simulink model "Full_Car_Model"  (R2023b)
settings: Solver=FixedStepAuto  StartTime=0.0  StopTime=t_end_sim  FixedStep=Ts_sim  RelTol=1e-3
values from neighbouring files (symbols this model uses):
  a_b_ref_sat = [ zeros(1,10) ... (first row only)    [A1_Init.m]    (also in C1_MonteCarloAnalysis.m)
  adaptive = 3    [A1_Init.m]    (also in C1_MonteCarloAnalysis.m = 1)
  data = A2_Full_car_model_parameters_4onBoard()    [A1_Init.m]    (also in C1_MonteCarloAnalysis.m)
  Ft_demand_F = [zeros(1,601) 200*ones(1,2400)]./data.R_F    [A1_Init.m]    (also in C1_MonteCarloAnalysis.m)
  Ft_demand_R = [zeros(1,(601-length(l_discr)))              200*ones(1,(2400+length(l_discr)))]./data.R_R    [A1_Init.m]    (also in C1_MonteCarloAnalysis.m)
  handmade_front = strcat(currentPath,'\Road_profiles\height_crg_files\','handmade_step_3cm_singlefunctions.crg')    [A1_Init.m]    (also in C1_MonteCarloAnalysis.m)
  handmade_mu_front = strcat(currentPath,'\Road_profiles\friction_crg_files\','handmade_fric_step_01_singlefunctions.crg')    [A1_Init.m]    (also in C1_MonteCarloAnalysis.m)
  handmade_mu_rear = handmade_mu_front    [A1_Init.m]    (also in C1_MonteCarloAnalysis.m)
  handmade_rear = handmade_front    [A1_Init.m]    (also in C1_MonteCarloAnalysis.m)
  LowLim_Q1 = -10    [A1_Init.m]    (also in C1_MonteCarloAnalysis.m)
  M = N    (= 10)    [A1_Init.m]    (also in C1_MonteCarloAnalysis.m)
  mu_distance = test_distance    [A1_Init.m]    (also in C1_MonteCarloAnalysis.m)
  mu_road = [ones(1,1001), 0.1*ones(1,2000)]    [A1_Init.m]    (also in C1_MonteCarloAnalysis.m)
  N = 10    [A1_Init.m]    (also in C1_MonteCarloAnalysis.m)
  N_iter = 3    [A1_Init.m]    (also in C1_MonteCarloAnalysis.m)
  omega_ini_F_L = x_u_dot_ini_F_L/data.R_F    [A1_Init.m]    (also in C1_MonteCarloAnalysis.m)
  omega_ini_F_R = x_u_dot_ini_R_R/data.R_F    [A1_Init.m]    (also in C1_MonteCarloAnalysis.m)
  omega_ini_R_L = x_u_dot_ini_R_L/data.R_R +2.483*1e-6    [A1_Init.m]    (also in C1_MonteCarloAnalysis.m)
  omega_ini_R_R = x_u_dot_ini_R_R/data.R_R+2.483*1e-6    [A1_Init.m]    (also in C1_MonteCarloAnalysis.m)
  passive = 2    [A1_Init.m]    (also in C1_MonteCarloAnalysis.m)
  Pitch = 0    [A1_Init.m]    (also in C1_MonteCarloAnalysis.m)
  Pitch_dot = 0    [A1_Init.m]    (also in C1_MonteCarloAnalysis.m)
  preview = 2    [A1_Init.m]    (also in C1_MonteCarloAnalysis.m)
  Q1 = 1e6    (= 1000000)    [A1_Init.m]    (also in C1_MonteCarloAnalysis.m)
  Q1_sat = 0    [A1_Init.m]    (also in C1_MonteCarloAnalysis.m)
  Q2 = 1e5    (= 100000)    [A1_Init.m]    (also in C1_MonteCarloAnalysis.m)
  QN1 = 0    [A1_Init.m]    (also in C1_MonteCarloAnalysis.m)
  QN2 = 0    [A1_Init.m]    (also in C1_MonteCarloAnalysis.m)
  R1 = 1e10    (= 10000000000)    [A1_Init.m]    (also in C1_MonteCarloAnalysis.m)
  r1_h0 = 0.99    [A1_Init.m]    (also in C1_MonteCarloAnalysis.m)
  r1_k = 1000    [A1_Init.m]    (also in C1_MonteCarloAnalysis.m)
  r1_max = 11    [A1_Init.m]    (also in C1_MonteCarloAnalysis.m)
  r1_min = -10    [A1_Init.m]    (also in C1_MonteCarloAnalysis.m)
  r2 = 2    [A1_Init.m]    (also in C1_MonteCarloAnalysis.m)
  R2 = 1e2    (= 100)    [A1_Init.m]    (also in C1_MonteCarloAnalysis.m)
  R2_rl = 2    [A1_Init.m]    (also in C1_MonteCarloAnalysis.m)
  road_profile = [zeros(1,801),ones(1,2200)*10*Step_selector]    [A1_Init.m]    (also in C1_MonteCarloAnalysis.m)
  T_distance = test_distance    [A1_Init.m]    (also in C1_MonteCarloAnalysis.m)
  T_hs_ini_F_L = 0    [A1_Init.m]    (also in C1_MonteCarloAnalysis.m)
  T_hs_ini_F_R = 0    [A1_Init.m]    (also in C1_MonteCarloAnalysis.m)
  T_hs_ini_R_L = 0    [A1_Init.m]    (also in C1_MonteCarloAnalysis.m)
  T_hs_ini_R_R = 0    [A1_Init.m]    (also in C1_MonteCarloAnalysis.m)
  test_distance = 0:0.01:30    [A1_Init.m]    (also in C1_MonteCarloAnalysis.m)
  theta_s_ini_F_L = 0    [A1_Init.m]    (also in C1_MonteCarloAnalysis.m)
  theta_s_ini_F_R = 0    [A1_Init.m]    (also in C1_MonteCarloAnalysis.m)
  theta_s_ini_R_L = 0    [A1_Init.m]    (also in C1_MonteCarloAnalysis.m)
  theta_s_ini_R_R = 0    [A1_Init.m]    (also in C1_MonteCarloAnalysis.m)
  theta_w_ini_F_L = -1.056*1e-2    (= -0.01056)    [A1_Init.m]    (also in C1_MonteCarloAnalysis.m)
  theta_w_ini_R_L = -1.056*1e-2    (= -0.01056)    [A1_Init.m]    (also in C1_MonteCarloAnalysis.m)
  Ts = 1e-3*[0 5 10 15 20 25 30 40 60 80 100]    [A1_Init.m]    (also in C1_MonteCarloAnalysis.m)
  w1_h0 = 0.0008    [A1_Init.m]    (also in C1_MonteCarloAnalysis.m)
  w1_k = 5000    [A1_Init.m]    (also in C1_MonteCarloAnalysis.m)
  w1_max = 9    [A1_Init.m]    (also in C1_MonteCarloAnalysis.m)
  w1_min = -10    [A1_Init.m]    (also in C1_MonteCarloAnalysis.m)
  w1_sat = 0.085    [A1_Init.m]    (also in C1_MonteCarloAnalysis.m)
  w2_h0 = 2    [A1_Init.m]    (also in C1_MonteCarloAnalysis.m)
  w2_inc = 0.05    [A1_Init.m]    (also in C1_MonteCarloAnalysis.m)
  w2_k = 10    [A1_Init.m]    (also in C1_MonteCarloAnalysis.m)
  w2_max = 5.3    [A1_Init.m]    (also in C1_MonteCarloAnalysis.m)
  w2_min = -10    [A1_Init.m]    (also in C1_MonteCarloAnalysis.m)
  Wmat_NMPC_init = [W(1,:) W(2,:) W(3,:) W(4,:)]    [A1_Init.m]    (also in C1_MonteCarloAnalysis.m)
  WNmat_NMPC_init = [WN(1,:) WN(2,:)]    [A1_Init.m]    (also in C1_MonteCarloAnalysis.m)
  X_0 = [z_b_dot_ini z_b_ini z_u_dot_ini_F_L z_u_ini_F_L x_b_dot_ini x_b_ini x_u_dot_ini_F_L x_u_ini_F_L          omega_ini_F_L theta_w_ini_F_L omega_ini_F_L theta_s_ini_F_L torque_ini_F_L]    [A1_Init.m]    (also in C1_MonteCarloAnalysis.m)
  x_b_dot_ini = speed_ini/3.6    (= 11.1111111111)    [A1_Init.m]    (also in C1_MonteCarloAnalysis.m)
  x_b_ini = data.b+pos_ini    [A1_Init.m]    (also in C1_MonteCarloAnalysis.m)
  x_u_dot_ini_F_L = speed_ini/3.6 - 1.125*1e-4    (= 11.1109986111)    [A1_Init.m]    (also in C1_MonteCarloAnalysis.m)
  x_u_dot_ini_F_R = speed_ini/3.6 - 1.125*1e-4    (= 11.1109986111)    [A1_Init.m]    (also in C1_MonteCarloAnalysis.m)
  x_u_dot_ini_R_L = speed_ini/3.6 - 1.125*1e-4    (= 11.1109986111)    [A1_Init.m]    (also in C1_MonteCarloAnalysis.m)
  x_u_dot_ini_R_R = speed_ini/3.6 - 1.125*1e-4    (= 11.1109986111)    [A1_Init.m]    (also in C1_MonteCarloAnalysis.m)
  x_u_ini_F_L = data.a+data.b+pos_ini    [A1_Init.m]    (also in C1_MonteCarloAnalysis.m)
  x_u_ini_F_R = data.a+data.b+pos_ini    [A1_Init.m]    (also in C1_MonteCarloAnalysis.m)
  x_u_ini_R_L = pos_ini    (= 0)    [A1_Init.m]    (also in C1_MonteCarloAnalysis.m)
  x_u_ini_R_R = pos_ini    (= 0)    [A1_Init.m]    (also in C1_MonteCarloAnalysis.m)
  z_b_dot_ini = 0    [A1_Init.m]    (also in C1_MonteCarloAnalysis.m)
  z_b_ini = 0    [A1_Init.m]    (also in C1_MonteCarloAnalysis.m)
  z_u_dot_ini_F_L = 0    [A1_Init.m]    (also in C1_MonteCarloAnalysis.m)
  z_u_dot_ini_F_R = 0    [A1_Init.m]    (also in C1_MonteCarloAnalysis.m)
  z_u_dot_ini_R_L = 0    [A1_Init.m]    (also in C1_MonteCarloAnalysis.m)
  z_u_dot_ini_R_R = 0    [A1_Init.m]    (also in C1_MonteCarloAnalysis.m)
  z_u_ini_F_L = 0    [A1_Init.m]    (also in C1_MonteCarloAnalysis.m)
  z_u_ini_F_R = 0    [A1_Init.m]    (also in C1_MonteCarloAnalysis.m)
  z_u_ini_R_L = 0    [A1_Init.m]    (also in C1_MonteCarloAnalysis.m)
  z_u_ini_R_R = 0    [A1_Init.m]    (also in C1_MonteCarloAnalysis.m)
undefined symbols (not defined in the file or in its folder): Delay_step, road_with_noise
libraries: mfswift_library x8, rllib x4, simulink x4
(part 4 of 7)

== system Full_Car_Model/PLANT MODEL WITH MF-SWIFT/REAR RIGHT WHEEL ==
  note: Rear rotational balance
  Tt_R_R : Inport
  BUS : Inport  Port=2
  Add1 : Sum
  Bus Creator : BusCreator  Inputs=3
  Bus Selector3 : BusSelector  OutputSignals=vertical_deflection,effective_rolling_radius,eff_plane_height,eff_plane_angle,longitudinal_slip,mu_x
  Clock1 : Clock
  Constant3 : Constant
  Demux1 : Demux  Outputs=2
  Gain3 : Gain  Gain=1/(data.I_y_R)
  Integrate velocity1 : Integrator  InitialCondition=theta_w_ini_R_L
  Integrate wheel acceleration : Integrator  InitialCondition=omega_ini_R_R
  MF-Swift : mfswift_library/MF-Swift  Tag=STI tyre  idtyre=2  tpfname=tir_name_R  rdfname=[handmade_rear,';',handmade_mu_rear];  road_mode=(2xxxx) opencrg  side_mode=(x3xxx) symmetric  cnt_mode=(xx5xx) enveloping  dyn_mode=(xxx3x) rigid-ring  mf_mode=(xxxx1) longitudinal  tv_model=Disabled  overwrite=off  use_mode=ISWITCH  internal_solver=off  enable_rr_init=on  optional_input=''  override_typarr=off  disp_debug=off
  "Select Fz, wheel" : Selector  InputPortWidth=3  IndexOptions=Index vector (dialog)  Indices=[1 3]  OutputSizes=[(-2)]
  Select My,wheel1 : Selector  InputPortWidth=3  IndexOptions=Index vector (dialog)  Indices=2  OutputSizes=[(-2)]
  Subsystem2 : Subsystem
  Subsystem5 : Subsystem
  Subsystem7 : Subsystem
  Terminator11 : Terminator
  Terminator13 : Terminator
  Terminator3 : Terminator
  To Workspace1 : ToWorkspace  VariableName=force_R_R  SampleTime=-1
  To Workspace4 : ToWorkspace  VariableName=torque_R_R  SampleTime=-1
  local2global : mfswift_library/local2global  Tag=local2global  init_pos=[0 0 (0.3833 - 0.5*data.m_total*9.81*data.a/data.L/data.k_t_R)]  init_angle=[0 0 0]
  Fx_R_R : Outport  VectorParamsAs1DForOutWhenUnconnected=off
  Fz_R_R_tot : Outport  Port=2  VectorParamsAs1DForOutWhenUnconnected=off
  Rotational_R_R : Outport  Port=3  VectorParamsAs1DForOutWhenUnconnected=off
  Slip_R_R : Outport  Port=4  VectorParamsAs1DForOutWhenUnconnected=off
  tag scope: mu_swift_R_R=global, w_swift_R_R=global
  wires:
  Demux1/1 -> Fx_R_R/1  "Fx_R_R"
  Bus Selector3/6 -> [mu_swift_R_R]  "<mu_x>"
  Bus Selector3/5 -> Slip_R_R/1  "<longitudinal_slip>"
  Gain3/1 -> Integrate wheel acceleration/1, Bus Creator/1  "omega_dot_R_R"
  Integrate wheel acceleration/1 -> Integrate velocity1/1, Bus Creator/2, MF-Swift/6  "omega_R_R"
  Bus Creator/1 -> Rotational_R_R/1
  Integrate velocity1/1 -> Bus Creator/3, MF-Swift/3  "theta_R_R"
  local2global/1 -> MF-Swift/1
  "Select Fz, wheel"/1 -> Demux1/1
  Tt_R_R/1 -> Add1/1
  Add1/1 -> Gain3/1
  Subsystem7/1(Road) -> MF-Swift/7  "With enveloping model i don't need this input"
  Bus Selector3/2 -> Terminator3/1  "<effective_rolling_radius>"
  MF-Swift/1 -> To Workspace1/1, "Select Fz, wheel"/1
  Constant3/1 -> Subsystem7/2(gain)
  Subsystem2/1(Velocity) -> local2global/1, MF-Swift/4
  MF-Swift/2 -> To Workspace4/1, Select My,wheel1/1
  MF-Swift/3 -> Bus Selector3/1
  Bus Selector3/1 -> Terminator13/1  "<vertical_deflection>"
  Demux1/2 -> Fz_R_R_tot/1
  Bus Selector3/4 -> Terminator11/1  "<eff_plane_angle>"
  Clock1/1 -> Subsystem7/1(time)
  local2global/2 -> MF-Swift/2
  Bus Selector3/3 -> [w_swift_R_R]  "<eff_plane_height>"
  Select My,wheel1/1 -> Add1/2
  Subsystem5/1(AngularVelocity) -> local2global/2, MF-Swift/5
  BUS/1 -> Subsystem2/1(speed), Subsystem5/1(Angular Speed)

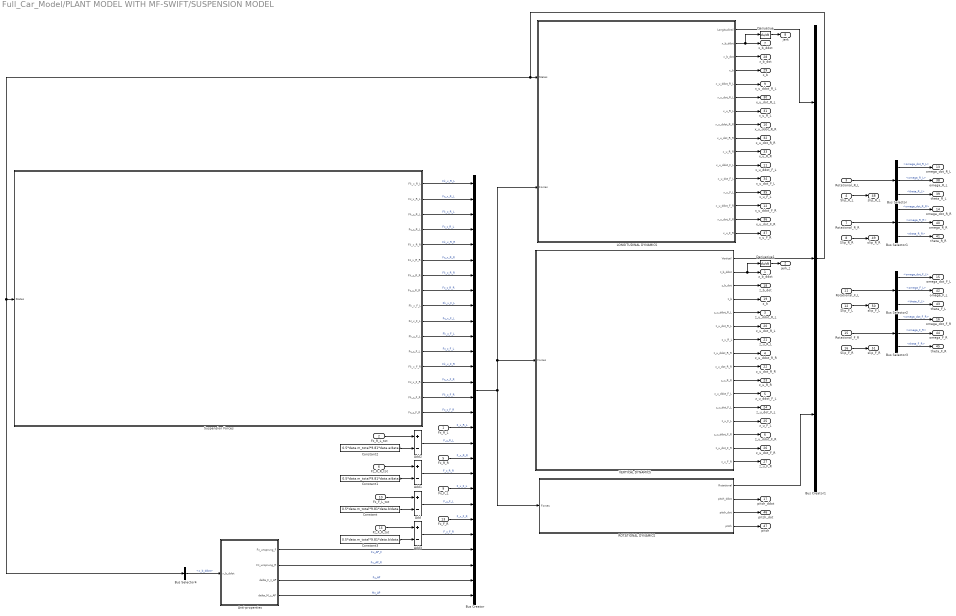
== system Full_Car_Model/PLANT MODEL WITH MF-SWIFT/SUSPENSION MODEL ==
  Fx_R_L : Inport
  Fz_R_L_tot : Inport  Port=2
  Rotational_R_L : Inport  Port=3
  Slip_R_L : Inport  Port=4
  Fx_R_R : Inport  Port=5
  Fz_R_R_tot : Inport  Port=6
  Rotational_R_R : Inport  Port=7
  Slip_R_R : Inport  Port=8
  Fx_F_L : Inport  Port=9
  Fz_F_L_tot : Inport  Port=10
  Rotational_F_L : Inport  Port=11
  Slip_F_L : Inport  Port=12
  Fx_F_R : Inport  Port=13
  Fz_F_R_tot : Inport  Port=14
  Rotational_F_R : Inport  Port=15
  Slip_F_R : Inport  Port=16
  Add{,1..3} (4 alike) : Sum  Inputs=+-
  Anti-properties : MATLAB Function  TreatAsAtomicUnit=on
  Bus Creator : BusCreator  Inputs=28
  Bus Creator1 : BusCreator  Inputs=3
  Bus Selector : BusSelector  OutputSignals=omega_dot_R_L,omega_R_L,theta_R_L
  Bus Selector1 : BusSelector  OutputSignals=omega_dot_R_R,omega_R_R,theta_R_R
  Bus Selector2 : BusSelector  OutputSignals=omega_dot_F_L,omega_F_L,theta_F_L
  Bus Selector3 : BusSelector  OutputSignals=omega_dot_F_R,omega_F_R,theta_F_R
  Bus Selector4 : BusSelector  OutputSignals=Longitudinal.x_b_ddot
  Constant : Constant  Value=0.5*data.m_total*9.81*data.b/data.L
  Constant1 : Constant  Value=0.5*data.m_total*9.81*data.a/data.L
  Constant2 : Constant  Value=0.5*data.m_total*9.81*data.a/data.L
  Constant3 : Constant  Value=0.5*data.m_total*9.81*data.b/data.L
  Derivative : Derivative
  Derivative1 : Derivative
  LONGITUDINAL DYNAMICS : Subsystem
  ROTATIONAL DYNAMICS : Subsystem
  Suspension Forces : Subsystem
  VERTICAL DYNAMICS : Subsystem
  z_b_ddot : Outport
  jerk_z : Outport  Port=2
  z_u_ddot_R_L : Outport  Port=3
  z_u_ddot_R_R : Outport  Port=4
  z_u_ddot_F_L : Outport  Port=5
  z_u_ddot_F_R : Outport  Port=6
  x_b_ddot : Outport  Port=7
  jerk : Outport  Port=8
  x_u_ddot_R_L : Outport  Port=9
  x_u_ddot_R_R : Outport  Port=10
  x_u_ddot_F_L : Outport  Port=11
  x_u_ddot_F_R : Outport  Port=12
  omega_dot_R_L : Outport  Port=13
  omega_dot_R_R : Outport  Port=14
  omega_dot_F_L : Outport  Port=15
  omega_dot_F_R : Outport  Port=16
  pitch_ddot : Outport  Port=17
  z_b_dot : Outport  Port=18
  z_b : Outport  Port=19
  z_u_dot_R_L : Outport  Port=20
  z_u_R_L : Outport  Port=21
  z_u_dot_R_R : Outport  Port=22
  z_u_R_R : Outport  Port=23
  z_u_dot_F_L : Outport  Port=24
  z_u_F_L : Outport  Port=25
  z_u_dot_F_R : Outport  Port=26
  z_u_F_R : Outport  Port=27
  x_b_dot : Outport  Port=28
  x_b : Outport  Port=29
  x_u_dot_R_L : Outport  Port=30
  x_u_R_L : Outport  Port=31
  x_u_dot_R_R : Outport  Port=32
  x_u_R_R : Outport  Port=33
  x_u_dot_F_L : Outport  Port=34
  x_u_F_L : Outport  Port=35
  x_u_dot_F_R : Outport  Port=36
  x_u_F_R : Outport  Port=37
  omega_R_L : Outport  Port=38
  theta_R_L : Outport  Port=39
  omega_R_R : Outport  Port=40
  theta_R_R : Outport  Port=41
  omega_F_L : Outport  Port=42
  theta_F_L : Outport  Port=43
  omega_F_R : Outport  Port=44
  theta_F_R : Outport  Port=45
  pitch_dot : Outport  Port=46
  pitch : Outport  Port=47
  slip_R_L : Outport  Port=48
  slip_R_R : Outport  Port=49
  slip_F_L : Outport  Port=50
  slip_F_R : Outport  Port=51
  wires:
  Anti-properties/2(Fz_unsprung_R) -> Bus Creator/26  "Fu_AP_R"
  Bus Selector4/1 -> Anti-properties/1(x_b_ddot)  "<x_b_ddot>"
  Anti-properties/4(delta_M_z_AP) -> Bus Creator/28  "Mz_AP"
  Anti-properties/3(delta_F_z_AP) -> Bus Creator/27  "Fz_AP"
  Anti-properties/1(Fz_unsprung_F) -> Bus Creator/25  "Fu_AP_F"
  Bus Creator1/1 -> LONGITUDINAL DYNAMICS/1(States), Suspension Forces/1(States), Bus Selector4/1
  Derivative1/1 -> jerk_z/1
  Derivative/1 -> jerk/1
  Slip_F_R/1 -> slip_F_R/1
  Bus Selector3/1 -> omega_dot_F_R/1  "<omega_dot_F_R>"
  Bus Selector3/2 -> omega_F_R/1  "<omega_F_R>"
  Bus Selector3/3 -> theta_F_R/1  "<theta_F_R>"
  Slip_F_L/1 -> slip_F_L/1
  Bus Selector2/3 -> theta_F_L/1  "<theta_F_L>"
  Bus Selector2/2 -> omega_F_L/1  "<omega_F_L>"
  Bus Selector2/1 -> omega_dot_F_L/1  "<omega_dot_F_L>"
  Slip_R_R/1 -> slip_R_R/1
  Bus Selector1/1 -> omega_dot_R_R/1  "<omega_dot_R_R>"
  Bus Selector1/2 -> omega_R_R/1  "<omega_R_R>"
  Bus Selector1/3 -> theta_R_R/1  "<theta_R_R>"
  Slip_R_L/1 -> slip_R_L/1
  Bus Selector/3 -> theta_R_L/1  "<theta_R_L>"
  Bus Selector/2 -> omega_R_L/1  "<omega_R_L>"
  Bus Selector/1 -> omega_dot_R_L/1  "<omega_dot_R_L>"
  Rotational_F_R/1 -> Bus Selector3/1
  Rotational_F_L/1 -> Bus Selector2/1
  Rotational_R_R/1 -> Bus Selector1/1
  Rotational_R_L/1 -> Bus Selector/1
  VERTICAL DYNAMICS/2(z_b_ddot) -> z_b_ddot/1, Derivative1/1
  VERTICAL DYNAMICS/3(z_b_dot) -> z_b_dot/1
  VERTICAL DYNAMICS/7(z_u_R_L) -> z_u_R_L/1
  VERTICAL DYNAMICS/6(z_u_dot_R_L) -> z_u_dot_R_L/1
  VERTICAL DYNAMICS/5(z_u_ddot_R_L) -> z_u_ddot_R_L/1
  VERTICAL DYNAMICS/4(z_b) -> z_b/1
  VERTICAL DYNAMICS/10(z_u_R_R) -> z_u_R_R/1
  VERTICAL DYNAMICS/11(z_u_ddot_F_L) -> z_u_ddot_F_L/1
  VERTICAL DYNAMICS/12(z_u_dot_F_L) -> z_u_dot_F_L/1
  VERTICAL DYNAMICS/13(z_u_F_L) -> z_u_F_L/1
  VERTICAL DYNAMICS/9(z_u_dot_R_R) -> z_u_dot_R_R/1
  VERTICAL DYNAMICS/8(z_u_ddot_R_R) -> z_u_ddot_R_R/1
  VERTICAL DYNAMICS/16(z_u_F_R) -> z_u_F_R/1
  VERTICAL DYNAMICS/15(z_u_dot_F_R) -> z_u_dot_F_R/1
  VERTICAL DYNAMICS/14(z_u_ddot_F_R) -> z_u_ddot_F_R/1
  ROTATIONAL DYNAMICS/2(pitch_ddot) -> pitch_ddot/1
  ROTATIONAL DYNAMICS/4(pitch) -> pitch/1
  ROTATIONAL DYNAMICS/3(pitch_dot) -> pitch_dot/1
  LONGITUDINAL DYNAMICS/14(x_u_ddot_F_R) -> x_u_ddot_F_R/1
  LONGITUDINAL DYNAMICS/15(x_u_dot_F_R) -> x_u_dot_F_R/1
  LONGITUDINAL DYNAMICS/16(x_u_F_R) -> x_u_F_R/1
  LONGITUDINAL DYNAMICS/8(x_u_ddot_R_R) -> x_u_ddot_R_R/1
  LONGITUDINAL DYNAMICS/9(x_u_dot_R_R) -> x_u_dot_R_R/1
  LONGITUDINAL DYNAMICS/13(x_u_F_L) -> x_u_F_L/1
  LONGITUDINAL DYNAMICS/12(x_u_dot_F_L) -> x_u_dot_F_L/1
  LONGITUDINAL DYNAMICS/11(x_u_ddot_F_L) -> x_u_ddot_F_L/1
  LONGITUDINAL DYNAMICS/10(x_u_R_R) -> x_u_R_R/1
  LONGITUDINAL DYNAMICS/4(x_b) -> x_b/1
  LONGITUDINAL DYNAMICS/5(x_u_ddot_R_L) -> x_u_ddot_R_L/1
  LONGITUDINAL DYNAMICS/6(x_u_dot_R_L) -> x_u_dot_R_L/1
  LONGITUDINAL DYNAMICS/7(x_u_R_L) -> x_u_R_L/1
  LONGITUDINAL DYNAMICS/3(x_b_dot) -> x_b_dot/1
  LONGITUDINAL DYNAMICS/2(x_b_ddot) -> x_b_ddot/1, Derivative/1
  ROTATIONAL DYNAMICS/1(Rotational) -> Bus Creator1/3
  VERTICAL DYNAMICS/1(Vertical) -> Bus Creator1/2
  LONGITUDINAL DYNAMICS/1(Longitudinal) -> Bus Creator1/1
  Bus Creator/1 -> ROTATIONAL DYNAMICS/1(Forces), LONGITUDINAL DYNAMICS/2(Forces), VERTICAL DYNAMICS/1(Forces)
  Suspension Forces/2(Fc_x_R_L) -> Bus Creator/2  "Fc_x_R_L"
  Suspension Forces/3(Fk_z_R_L) -> Bus Creator/3  "Fk_z_R_L"
  Suspension Forces/4(Fc_z_R_L) -> Bus Creator/4  "Fc_z_R_L"
  Suspension Forces/5(Fk_x_R_R) -> Bus Creator/5  "Fk_x_R_R"
  Suspension Forces/6(Fc_x_R_R) -> Bus Creator/6  "Fc_x_R_R"
  Suspension Forces/7(Fk_z_R_R) -> Bus Creator/7  "Fk_z_R_R"
  Suspension Forces/8(Fc_z_R_R) -> Bus Creator/8  "Fc_z_R_R"
  Suspension Forces/9(Fk_x_F_L) -> Bus Creator/9  "Fk_x_F_L"
  Suspension Forces/10(Fc_x_F_L) -> Bus Creator/10  "Fc_x_F_L"
  Suspension Forces/11(Fk_z_F_L) -> Bus Creator/11  "Fk_z_F_L"
  Suspension Forces/12(Fc_z_F_L) -> Bus Creator/12  "Fc_z_F_L"
  Suspension Forces/13(Fk_x_F_R) -> Bus Creator/13  "Fk_x_F_R"
  Suspension Forces/14(Fc_x_F_R) -> Bus Creator/14  "Fc_x_F_R"
  Suspension Forces/15(Fk_z_F_R) -> Bus Creator/15  "Fk_z_F_R"
  Suspension Forces/16(Fc_z_F_R) -> Bus Creator/16  "Fc_z_F_R"
  Suspension Forces/1(Fk_x_R_L) -> Bus Creator/1  "Fk_x_R_L"
  Constant3/1 -> Add3/2
  Fz_F_R_tot/1 -> Add3/1
  Add3/1 -> Bus Creator/24  "F_z_F_R"
  Add1/1 -> Bus Creator/20  "F_z_R_R"
  Constant1/1 -> Add1/2
  Fz_R_R_tot/1 -> Add1/1
  Add2/1 -> Bus Creator/18  "F_z_R_L"
  Constant2/1 -> Add2/2
  Fz_R_L_tot/1 -> Add2/1
  Add/1 -> Bus Creator/22  "F_z_F_L"
  Constant/1 -> Add/2
  Fz_F_L_tot/1 -> Add/1
  Fx_R_L/1 -> Bus Creator/17  "F_x_R_L"
  Fx_R_R/1 -> Bus Creator/19  "F_x_R_R"
  Fx_F_L/1 -> Bus Creator/21  "F_x_F_L"
  Fx_F_R/1 -> Bus Creator/23  "F_x_F_R"

== system Full_Car_Model/CONTROLLER FRONT LEFT/RL_weights/Subsystem2 ==
  Online Data : Inport
  Delay : Delay  Commented=on  DelayLength=1  SampleTime=Ts(2)
  MATLAB Function : MATLAB Function  TreatAsAtomicUnit=on
  Memory{,1..4} (5 alike) : Memory  InheritSampleTime=on
  Mux : Mux  Inputs=5
  Mux2 : Mux  Inputs=2
  Selector : Selector  NumberOfDimensions=2  InputPortWidth=1  IndexOptions=Index vector (dialog),Select all  Indices=1,1  OutputSizes=1,1
  Selector1 : Selector  NumberOfDimensions=2  InputPortWidth=1  IndexOptions=Index vector (dialog),Select all  Indices=1,1  OutputSizes=1,1
  w_prev : Outport
  mu_act_prev : Outport  Port=2
  sigma_ref_act : Outport  Port=3
  wires:
  Online Data/1 -> MATLAB Function/1(OnlineData)
  MATLAB Function/1(w) -> Mux2/2, Selector/1
  Selector/1 -> Memory/1  "w1"
  Memory/1 -> Memory1/1, Mux/5
  Memory1/1 -> Memory2/1, Mux/4
  Memory2/1 -> Memory3/1, Mux/3
  Memory3/1 -> Memory4/1, Mux/2
  Memory4/1 -> Mux/1
  Mux/1 -> Mux2/1
  Mux2/1 -> w_prev/1
  MATLAB Function/2(mu_act) -> mu_act_prev/1
  MATLAB Function/3(sigma_ref) -> Selector1/1
  Selector1/1 -> sigma_ref_act/1

== system Full_Car_Model/CONTROLLER FRONT LEFT/ROAD PREVIEW/Time-based Road Preview ==
  note: Absolute longitudinal wheel position along t_h
      | (assuming contant speed along t_h)
  x_u : Inport
  x_u_dot : Inport  Port=2
  1-D Lookup Table : Lookup_n-D  NumberOfTableDimensions=1  BreakpointsForDimension1=mu_distance  Table=mu_road  InternalRulePriority=Speed  RndMeth=Simplest
  Delay1 : Delay  Commented=on  DelayLength=Delay_step
  Gain1 : Gain  Gain=1e-3
  MATLAB Function1 : MATLAB Function  TreatAsAtomicUnit=on
  MATLAB Function4 : MATLAB Function  TreatAsAtomicUnit=on
  MATLAB Function5 : MATLAB Function  TreatAsAtomicUnit=on
  To Workspace : ToWorkspace  VariableName=roadprofile_front_plot  SaveFormat=Timeseries  SampleTime=-1
  X(i)1 : MATLAB Function  TreatAsAtomicUnit=on
  Z_road with noise2 : Lookup_n-D  Commented=on  NumberOfTableDimensions=1  BreakpointsForDimension1=test_distance  Table=road_with_noise  InterpMethod=Flat  InternalRulePriority=Speed  RndMeth=Simplest
  Z_road1 : Lookup_n-D  NumberOfTableDimensions=1  BreakpointsForDimension1=test_distance  Table=road_profile  InterpMethod=Flat  InternalRulePriority=Speed  RndMeth=Simplest
  Z_road2 : Lookup_n-D  NumberOfTableDimensions=1  BreakpointsForDimension1=test_distance  Table=road_profile  InterpMethod=Flat  InternalRulePriority=Speed  RndMeth=Simplest
  w : Outport
  beta_y : Outport  Port=2
  mu_prev : Outport  Port=3
  wires:
  Z_road2/1 -> To Workspace/1
  MATLAB Function1/1(Z_ef) -> MATLAB Function4/1(Z_ef)
  MATLAB Function1/2(Z_er) -> MATLAB Function4/2(Z_er)
  1-D Lookup Table/1 -> mu_prev/1
  X(i)1/1(X_i) -> 1-D Lookup Table/1, MATLAB Function5/1(X_i)  "X(i)"
  Gain1/1 -> MATLAB Function1/1(z_road)
  MATLAB Function4/1(w) -> w/1
  Z_road1/1 -> Gain1/1
  MATLAB Function5/1(X_road) -> Z_road1/1
  x_u/1 -> X(i)1/1(X_u_current), Z_road2/1
  x_u_dot/1 -> X(i)1/2(x_u_dot_current)
  MATLAB Function4/2(beta_y) -> beta_y/1

== system Full_Car_Model/CONTROLLER FRONT LEFT/Rule based/Flag ==
  Measurement data : Inport
  mu_prev : Inport  Port=2
  Add : Sum  Inputs=+-
  Bus Selector : BusSelector  OutputSignals=Accelerations.x_b_ddot
  Constant : Constant  Value=0.5*data.m_total*data.g*data.b/data.L
  Gain : Gain  Gain=0.5*data.m_total*data.hg/data.L
  Gain1 : Gain  Gain=0.6
  GreaterThan : RelationalOperator  Operator=>  OutDataTypeStr=boolean  RndMeth=Simplest  InputSameDT=off
  Memory : Memory
  OR : Logic  Operator=OR  Inputs=1  IconShape=distinctive  AllPortsSameDT=off  OutDataTypeStr=boolean
  Product : Product
  Flag : Outport
  wires:
  Constant/1 -> Add/1
  Bus Selector/1 -> Memory/1  "<x_b_ddot>"
  [Ft_req_F] -> GreaterThan/1
  Gain/1 -> Add/2
  Add/1 -> Product/1
  Measurement data/1 -> Bus Selector/1
  GreaterThan/1 -> OR/1
  Product/1 -> Gain1/1
  Memory/1 -> Gain/1
  mu_prev/1 -> Product/2
  Gain1/1 -> GreaterThan/2
  OR/1 -> Flag/1

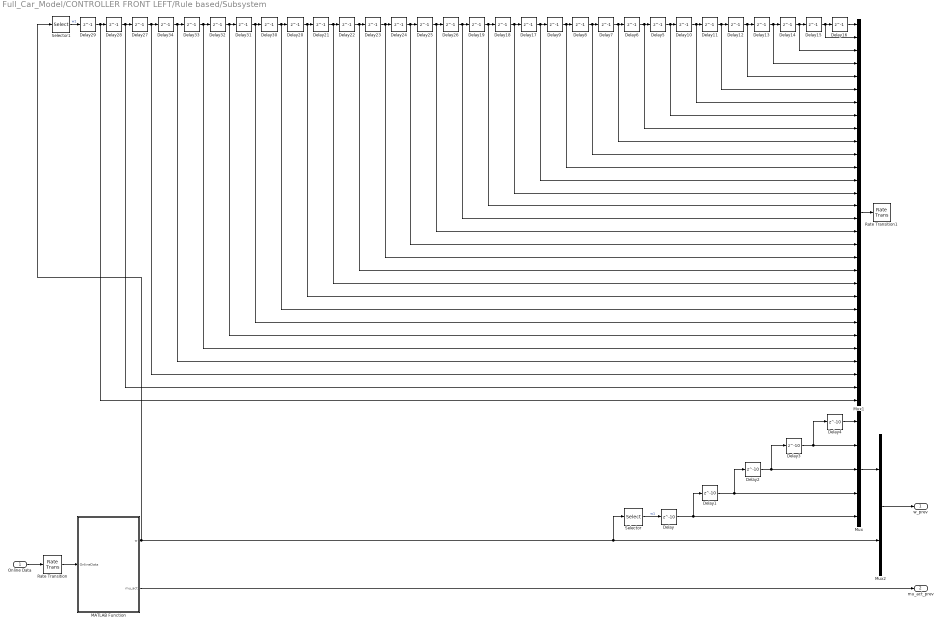
== system Full_Car_Model/CONTROLLER FRONT LEFT/Rule based/Subsystem ==
  Online Data : Inport
  Delay{,1..4} (5 alike) : Delay  DelayLength=10
  Delay{5..34} (30 alike) : Delay  DelayLength=1
  MATLAB Function : MATLAB Function  TreatAsAtomicUnit=on
  Mux : Mux  Inputs=5
  Mux1 : Mux  Inputs=30
  Mux2 : Mux  Inputs=2
  Rate Transition : RateTransition  OutPortSampleTime=Ts(2)
  Rate Transition1 : RateTransition  OutPortSampleTime=Ts(2)
  Selector : Selector  NumberOfDimensions=2  InputPortWidth=1  IndexOptions=Index vector (dialog),Select all  Indices=1,1  OutputSizes=1,1
  Selector1 : Selector  NumberOfDimensions=2  InputPortWidth=1  IndexOptions=Index vector (dialog),Select all  Indices=1,1  OutputSizes=1,1
  w_prev : Outport
  mu_act_prev : Outport  Port=2
  wires:
  MATLAB Function/1(w) -> Mux2/2, Selector/1, Selector1/1
  MATLAB Function/2(mu_act) -> mu_act_prev/1
  Mux1/1 -> Rate Transition1/1
  Rate Transition/1 -> MATLAB Function/1(OnlineData)
  Mux2/1 -> w_prev/1
  Delay4/1 -> Mux/1
  Delay3/1 -> Delay4/1, Mux/2
  Delay2/1 -> Delay3/1, Mux/3
  Delay1/1 -> Mux/4, Delay2/1
  Delay/1 -> Mux/5, Delay1/1
  Selector/1 -> Delay/1  "w1"
  Online Data/1 -> Rate Transition/1
  Delay5/1 -> Mux1/8, Delay10/1
  Selector1/1 -> Delay29/1  "w1"
  Delay10/1 -> Mux1/7, Delay11/1
  Delay11/1 -> Mux1/6, Delay12/1
  Delay12/1 -> Mux1/5, Delay13/1
  Delay13/1 -> Mux1/4, Delay14/1
  Delay14/1 -> Mux1/3, Delay15/1
  Delay15/1 -> Mux1/2, Delay16/1
  Delay16/1 -> Mux1/1
  Delay6/1 -> Mux1/9, Delay5/1
  Delay7/1 -> Mux1/10, Delay6/1
  Delay8/1 -> Delay7/1, Mux1/11
  Delay9/1 -> Mux1/12, Delay8/1
  Delay17/1 -> Mux1/13, Delay9/1
  Delay18/1 -> Mux1/14, Delay17/1
  Delay19/1 -> Delay18/1, Mux1/15
  Delay26/1 -> Mux1/16, Delay19/1
  Delay25/1 -> Mux1/17, Delay26/1
  Delay24/1 -> Mux1/18, Delay25/1
  Delay22/1 -> Mux1/20, Delay23/1
  Delay34/1 -> Mux1/27, Delay33/1
  Delay33/1 -> Mux1/26, Delay32/1
  Delay31/1 -> Mux1/24, Delay30/1
  Delay32/1 -> Mux1/25, Delay31/1
  Delay30/1 -> Mux1/23, Delay20/1
  Delay28/1 -> Mux1/29, Delay27/1
  Delay27/1 -> Mux1/28, Delay34/1
  Delay23/1 -> Mux1/19, Delay24/1
  Delay21/1 -> Mux1/21, Delay22/1
  Delay29/1 -> Mux1/30, Delay28/1
  Delay20/1 -> Mux1/22, Delay21/1
  Mux/1 -> Mux2/1

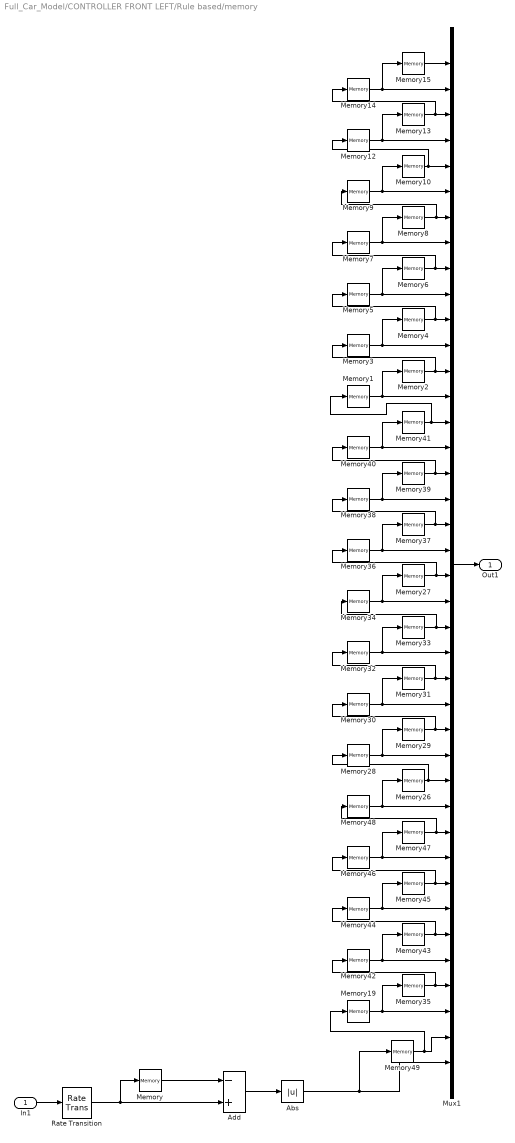
== system Full_Car_Model/CONTROLLER FRONT LEFT/Rule based/memory ==
  In1 : Inport
  Abs : Abs  SaturateOnIntegerOverflow=off
  Add : Sum  Inputs=-+
  Memory{,1..10,12..15,19,26..49} (40 alike) : Memory  InheritSampleTime=on
  Mux1 : Mux  Inputs=40
  Rate Transition : RateTransition  OutPortSampleTime=Ts(2)
  Out1 : Outport
  wires:
  Abs/1 -> Mux1/40, Memory49/1
  Memory49/1 -> Mux1/39, Memory19/1
  Memory19/1 -> Memory35/1, Mux1/38
  Memory47/1 -> Memory48/1, Mux1/31
  Memory42/1 -> Memory43/1, Mux1/36
  Memory44/1 -> Memory45/1, Mux1/34
  Memory43/1 -> Memory44/1, Mux1/35
  Memory33/1 -> Memory34/1, Mux1/23
  Memory46/1 -> Memory47/1, Mux1/32
  Memory32/1 -> Memory33/1, Mux1/24
  Memory38/1 -> Memory39/1, Mux1/18
  Memory48/1 -> Memory26/1, Mux1/30
  Memory45/1 -> Memory46/1, Mux1/33
  Memory30/1 -> Memory31/1, Mux1/26
  Memory26/1 -> Memory28/1, Mux1/29
  Memory37/1 -> Memory38/1, Mux1/19
  Memory29/1 -> Memory30/1, Mux1/27
  Memory31/1 -> Memory32/1, Mux1/25
  Memory27/1 -> Memory36/1, Mux1/21
  Memory28/1 -> Memory29/1, Mux1/28
  Memory34/1 -> Memory27/1, Mux1/22
  Memory40/1 -> Memory41/1, Mux1/16
  Memory41/1 -> Mux1/15, Memory1/1
  Memory39/1 -> Memory40/1, Mux1/17
  Memory35/1 -> Memory42/1, Mux1/37
  Memory36/1 -> Memory37/1, Mux1/20
  Add/1 -> Abs/1
  In1/1 -> Rate Transition/1
  Memory/1 -> Add/1
  Rate Transition/1 -> Add/2, Memory/1
  Memory14/1 -> Memory15/1, Mux1/2
  Memory12/1 -> Memory13/1, Mux1/4
  Memory15/1 -> Mux1/1
  Memory13/1 -> Memory14/1, Mux1/3
  Memory10/1 -> Mux1/5, Memory12/1
  Memory9/1 -> Memory10/1, Mux1/6
  Memory8/1 -> Memory9/1, Mux1/7
  Memory7/1 -> Memory8/1, Mux1/8
  Memory6/1 -> Memory7/1, Mux1/9
  Memory5/1 -> Memory6/1, Mux1/10
  Memory4/1 -> Mux1/11, Memory5/1
  Memory3/1 -> Memory4/1, Mux1/12
  Memory2/1 -> Mux1/13, Memory3/1
  Memory1/1 -> Memory2/1, Mux1/14
  Mux1/1 -> Out1/1

== system Full_Car_Model/CONTROLLER FRONT RIGHT/RL_weights/Subsystem2 ==
  Online Data : Inport
  Delay : Delay  Commented=on  DelayLength=1  SampleTime=Ts(2)
  MATLAB Function : MATLAB Function  TreatAsAtomicUnit=on
  Memory{,1..4} (5 alike) : Memory  InheritSampleTime=on
  Mux : Mux  Inputs=5
  Mux2 : Mux  Inputs=2
  Selector : Selector  NumberOfDimensions=2  InputPortWidth=1  IndexOptions=Index vector (dialog),Select all  Indices=1,1  OutputSizes=1,1
  Selector1 : Selector  NumberOfDimensions=2  InputPortWidth=1  IndexOptions=Index vector (dialog),Select all  Indices=1,1  OutputSizes=1,1
  w_prev : Outport
  mu_act_prev : Outport  Port=2
  sigma_ref_act : Outport  Port=3
  wires:
  Online Data/1 -> MATLAB Function/1(OnlineData)
  MATLAB Function/1(w) -> Mux2/2, Selector/1
  Selector/1 -> Memory/1  "w1"
  Memory/1 -> Memory1/1, Mux/5
  Memory1/1 -> Memory2/1, Mux/4
  Memory2/1 -> Memory3/1, Mux/3
  Memory3/1 -> Memory4/1, Mux/2
  Memory4/1 -> Mux/1
  Mux/1 -> Mux2/1
  Mux2/1 -> w_prev/1
  MATLAB Function/2(mu_act) -> mu_act_prev/1
  MATLAB Function/3(sigma_ref) -> Selector1/1
  Selector1/1 -> sigma_ref_act/1

== system Full_Car_Model/CONTROLLER FRONT RIGHT/ROAD PREVIEW/Time-based Road Preview ==
  note: Absolute longitudinal wheel position along t_h
      | (assuming contant speed along t_h)
  x_u : Inport
  x_u_dot : Inport  Port=2
  1-D Lookup Table : Lookup_n-D  NumberOfTableDimensions=1  BreakpointsForDimension1=mu_distance  Table=mu_road  InternalRulePriority=Speed  RndMeth=Simplest
  Delay1 : Delay  Commented=on  DelayLength=Delay_step
  Demux5 : Demux  Commented=on  Outputs=6
  Demux6 : Demux  Commented=on  Outputs=6
  Gain1 : Gain  Gain=1e-3
  Goto5 : Goto  Commented=on  GotoTag=beta_y_env_F_L  TagVisibility=global
  Goto6 : Goto  Commented=on  GotoTag=w_env_F_L  TagVisibility=global
  MATLAB Function2 : MATLAB Function  TreatAsAtomicUnit=on
  MATLAB Function3 : MATLAB Function  TreatAsAtomicUnit=on
  MATLAB Function6 : MATLAB Function  TreatAsAtomicUnit=on
  Terminator{1..7,20..22} (10 alike) : Terminator  Commented=on
  X(i)1 : MATLAB Function  TreatAsAtomicUnit=on
  Z_road with noise2 : Lookup_n-D  Commented=on  NumberOfTableDimensions=1  BreakpointsForDimension1=test_distance  Table=road_with_noise  InterpMethod=Flat  InternalRulePriority=Speed  RndMeth=Simplest
  Z_road1 : Lookup_n-D  NumberOfTableDimensions=1  BreakpointsForDimension1=test_distance  Table=road_profile  InterpMethod=Flat  InternalRulePriority=Speed  RndMeth=Simplest
  w : Outport
  beta_y : Outport  Port=2
  mu_prev : Outport  Port=3
  wires:
  Demux6/1 -> Goto5/1
  Demux6/5 -> Terminator7/1
  Demux6/2 -> Terminator5/1
  Demux6/3 -> Terminator6/1
  Demux6/6 -> Terminator3/1
  Demux6/4 -> Terminator4/1
  Demux5/4 -> Terminator2/1
  Demux5/5 -> Terminator22/1
  Demux5/6 -> Terminator1/1
  Demux5/3 -> Terminator21/1
  Demux5/2 -> Terminator20/1
  Demux5/1 -> Goto6/1
  MATLAB Function3/2(beta_y) -> beta_y/1, Demux6/1
  x_u_dot/1 -> X(i)1/2(x_u_dot_current)
  x_u/1 -> X(i)1/1(X_u_current)
  MATLAB Function6/1(X_road) -> Z_road1/1
  Z_road1/1 -> Gain1/1
  MATLAB Function3/1(w) -> Demux5/1, w/1
  Gain1/1 -> MATLAB Function2/1(z_road)
  X(i)1/1(X_i) -> 1-D Lookup Table/1, MATLAB Function6/1(X_i)  "X(i)"
  1-D Lookup Table/1 -> mu_prev/1
  MATLAB Function2/2(Z_er) -> MATLAB Function3/2(Z_er)
  MATLAB Function2/1(Z_ef) -> MATLAB Function3/1(Z_ef)

== system Full_Car_Model/CONTROLLER FRONT RIGHT/Rule based/Flag ==
  Measurement data : Inport
  mu_prev : Inport  Port=2
  Add : Sum  Inputs=+-
  Bus Selector : BusSelector  OutputSignals=Accelerations.x_b_ddot
  Constant : Constant  Value=0.5*data.m_total*data.g*data.b/data.L
  Gain : Gain  Gain=0.5*data.m_total*data.hg/data.L
  Gain1 : Gain  Gain=0.6
  GreaterThan : RelationalOperator  Operator=>  OutDataTypeStr=boolean  RndMeth=Simplest  InputSameDT=off
  Memory : Memory
  OR : Logic  Operator=OR  Inputs=1  IconShape=distinctive  AllPortsSameDT=off  OutDataTypeStr=boolean
  Product : Product
  Scope : Scope  NumInputPorts=3
  Flag : Outport
  wires:
  Constant/1 -> Add/1
  Bus Selector/1 -> Memory/1  "<x_b_ddot>"
  [Ft_req_F] -> Scope/1, GreaterThan/1
  Gain/1 -> Add/2
  Add/1 -> Product/1
  Measurement data/1 -> Bus Selector/1
  GreaterThan/1 -> Scope/3, OR/1
  Product/1 -> Gain1/1
  Memory/1 -> Gain/1
  mu_prev/1 -> Product/2
  Gain1/1 -> Scope/2, GreaterThan/2
  OR/1 -> Flag/1

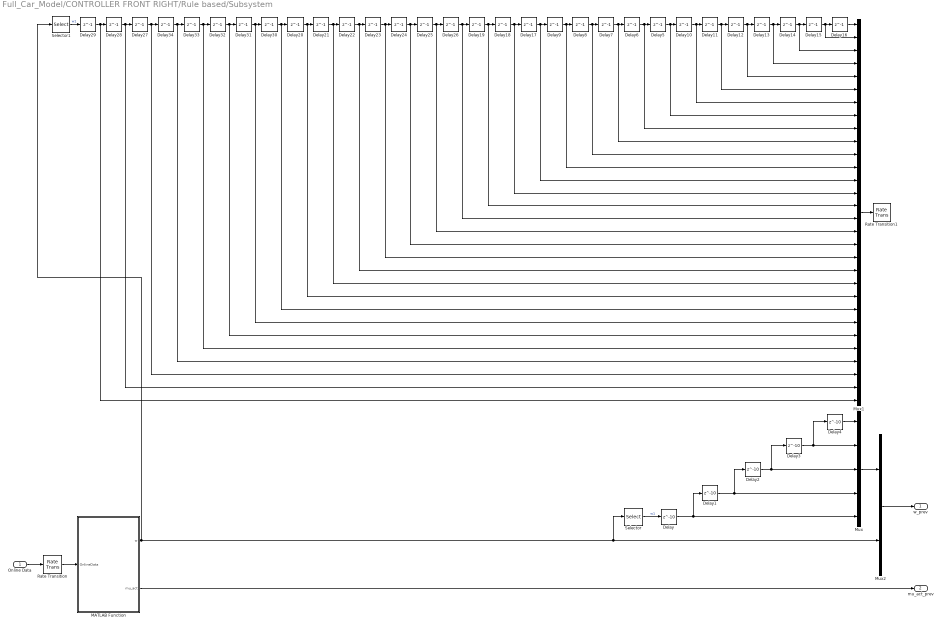
== system Full_Car_Model/CONTROLLER FRONT RIGHT/Rule based/Subsystem ==
  Online Data : Inport
  Delay{,1..4} (5 alike) : Delay  DelayLength=10
  Delay{5..34} (30 alike) : Delay  DelayLength=1
  MATLAB Function : MATLAB Function  TreatAsAtomicUnit=on
  Mux : Mux  Inputs=5
  Mux1 : Mux  Inputs=30
  Mux2 : Mux  Inputs=2
  Rate Transition : RateTransition  OutPortSampleTime=Ts(2)
  Rate Transition1 : RateTransition  OutPortSampleTime=Ts(2)
  Selector : Selector  NumberOfDimensions=2  InputPortWidth=1  IndexOptions=Index vector (dialog),Select all  Indices=1,1  OutputSizes=1,1
  Selector1 : Selector  NumberOfDimensions=2  InputPortWidth=1  IndexOptions=Index vector (dialog),Select all  Indices=1,1  OutputSizes=1,1
  w_prev : Outport
  mu_act_prev : Outport  Port=2
  wires:
  MATLAB Function/1(w) -> Mux2/2, Selector/1, Selector1/1
  MATLAB Function/2(mu_act) -> mu_act_prev/1
  Mux1/1 -> Rate Transition1/1
  Rate Transition/1 -> MATLAB Function/1(OnlineData)
  Mux2/1 -> w_prev/1
  Delay4/1 -> Mux/1
  Delay3/1 -> Delay4/1, Mux/2
  Delay2/1 -> Delay3/1, Mux/3
  Delay1/1 -> Mux/4, Delay2/1
  Delay/1 -> Mux/5, Delay1/1
  Selector/1 -> Delay/1  "w1"
  Online Data/1 -> Rate Transition/1
  Delay5/1 -> Mux1/8, Delay10/1
  Selector1/1 -> Delay29/1  "w1"
  Delay10/1 -> Mux1/7, Delay11/1
  Delay11/1 -> Mux1/6, Delay12/1
  Delay12/1 -> Mux1/5, Delay13/1
  Delay13/1 -> Mux1/4, Delay14/1
  Delay14/1 -> Mux1/3, Delay15/1
  Delay15/1 -> Mux1/2, Delay16/1
  Delay16/1 -> Mux1/1
  Delay6/1 -> Mux1/9, Delay5/1
  Delay7/1 -> Mux1/10, Delay6/1
  Delay8/1 -> Delay7/1, Mux1/11
  Delay9/1 -> Mux1/12, Delay8/1
  Delay17/1 -> Mux1/13, Delay9/1
  Delay18/1 -> Mux1/14, Delay17/1
  Delay19/1 -> Delay18/1, Mux1/15
  Delay26/1 -> Mux1/16, Delay19/1
  Delay25/1 -> Mux1/17, Delay26/1
  Delay24/1 -> Mux1/18, Delay25/1
  Delay22/1 -> Mux1/20, Delay23/1
  Delay34/1 -> Mux1/27, Delay33/1
  Delay33/1 -> Mux1/26, Delay32/1
  Delay31/1 -> Mux1/24, Delay30/1
  Delay32/1 -> Mux1/25, Delay31/1
  Delay30/1 -> Mux1/23, Delay20/1
  Delay28/1 -> Mux1/29, Delay27/1
  Delay27/1 -> Mux1/28, Delay34/1
  Delay23/1 -> Mux1/19, Delay24/1
  Delay21/1 -> Mux1/21, Delay22/1
  Delay29/1 -> Mux1/30, Delay28/1
  Delay20/1 -> Mux1/22, Delay21/1
  Mux/1 -> Mux2/1

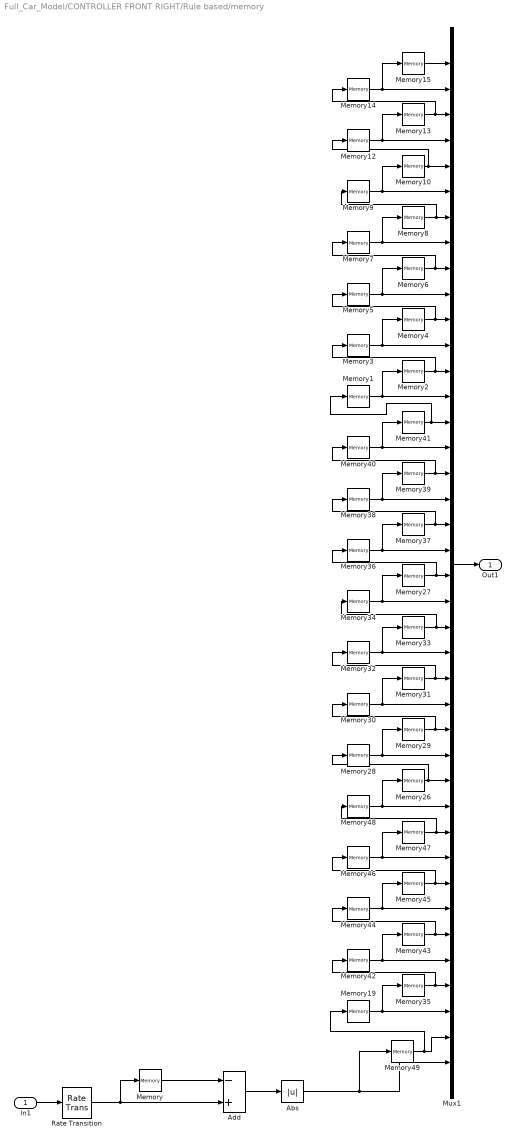
== system Full_Car_Model/CONTROLLER FRONT RIGHT/Rule based/memory ==
  In1 : Inport
  Abs : Abs  SaturateOnIntegerOverflow=off
  Add : Sum  Inputs=-+
  Memory{,1..10,12..15,19,26..49} (40 alike) : Memory  InheritSampleTime=on
  Mux1 : Mux  Inputs=40
  Rate Transition : RateTransition  OutPortSampleTime=Ts(2)
  Out1 : Outport
  wires:
  Abs/1 -> Mux1/40, Memory49/1
  Memory49/1 -> Mux1/39, Memory19/1
  Memory19/1 -> Memory35/1, Mux1/38
  Memory47/1 -> Memory48/1, Mux1/31
  Memory42/1 -> Memory43/1, Mux1/36
  Memory44/1 -> Memory45/1, Mux1/34
  Memory43/1 -> Memory44/1, Mux1/35
  Memory33/1 -> Memory34/1, Mux1/23
  Memory46/1 -> Memory47/1, Mux1/32
  Memory32/1 -> Memory33/1, Mux1/24
  Memory38/1 -> Memory39/1, Mux1/18
  Memory48/1 -> Memory26/1, Mux1/30
  Memory45/1 -> Memory46/1, Mux1/33
  Memory30/1 -> Memory31/1, Mux1/26
  Memory26/1 -> Memory28/1, Mux1/29
  Memory37/1 -> Memory38/1, Mux1/19
  Memory29/1 -> Memory30/1, Mux1/27
  Memory31/1 -> Memory32/1, Mux1/25
  Memory27/1 -> Memory36/1, Mux1/21
  Memory28/1 -> Memory29/1, Mux1/28
  Memory34/1 -> Memory27/1, Mux1/22
  Memory40/1 -> Memory41/1, Mux1/16
  Memory41/1 -> Mux1/15, Memory1/1
  Memory39/1 -> Memory40/1, Mux1/17
  Memory35/1 -> Memory42/1, Mux1/37
  Memory36/1 -> Memory37/1, Mux1/20
  Add/1 -> Abs/1
  In1/1 -> Rate Transition/1
  Memory/1 -> Add/1
  Rate Transition/1 -> Add/2, Memory/1
  Memory14/1 -> Memory15/1, Mux1/2
  Memory12/1 -> Memory13/1, Mux1/4
  Memory15/1 -> Mux1/1
  Memory13/1 -> Memory14/1, Mux1/3
  Memory10/1 -> Mux1/5, Memory12/1
  Memory9/1 -> Memory10/1, Mux1/6
  Memory8/1 -> Memory9/1, Mux1/7
  Memory7/1 -> Memory8/1, Mux1/8
  Memory6/1 -> Memory7/1, Mux1/9
  Memory5/1 -> Memory6/1, Mux1/10
  Memory4/1 -> Mux1/11, Memory5/1
  Memory3/1 -> Memory4/1, Mux1/12
  Memory2/1 -> Mux1/13, Memory3/1
  Memory1/1 -> Memory2/1, Mux1/14
  Mux1/1 -> Out1/1

== system Full_Car_Model/CONTROLLER REAR LEFT/RL_weights/Subsystem2 ==
  Online Data : Inport
  Delay : Delay  Commented=on  DelayLength=1  SampleTime=Ts(2)
  MATLAB Function : MATLAB Function  TreatAsAtomicUnit=on
  Memory{,1..4} (5 alike) : Memory  InheritSampleTime=on
  Mux : Mux  Inputs=5
  Mux2 : Mux  Inputs=2
  Selector : Selector  NumberOfDimensions=2  InputPortWidth=1  IndexOptions=Index vector (dialog),Select all  Indices=1,1  OutputSizes=1,1
  Selector1 : Selector  NumberOfDimensions=2  InputPortWidth=1  IndexOptions=Index vector (dialog),Select all  Indices=1,1  OutputSizes=1,1
  w_prev : Outport
  mu_act_prev : Outport  Port=2
  sigma_ref_act : Outport  Port=3
  wires:
  Online Data/1 -> MATLAB Function/1(OnlineData)
  MATLAB Function/1(w) -> Mux2/2, Selector/1
  Selector/1 -> Memory/1  "w1"
  Memory/1 -> Memory1/1, Mux/5
  Memory1/1 -> Memory2/1, Mux/4
  Memory2/1 -> Memory3/1, Mux/3
  Memory3/1 -> Memory4/1, Mux/2
  Memory4/1 -> Mux/1
  Mux/1 -> Mux2/1
  Mux2/1 -> w_prev/1
  MATLAB Function/2(mu_act) -> mu_act_prev/1
  MATLAB Function/3(sigma_ref) -> Selector1/1
  Selector1/1 -> sigma_ref_act/1

== system Full_Car_Model/CONTROLLER REAR LEFT/ROAD PREVIEW/Time-based Road Preview ==
  note: Absolute longitudinal wheel position along t_h
      | (assuming contant speed along t_h)
  x_u : Inport
  x_u_dot : Inport  Port=2
  1-D Lookup Table : Lookup_n-D  NumberOfTableDimensions=1  BreakpointsForDimension1=mu_distance  Table=mu_road  InternalRulePriority=Speed  RndMeth=Simplest
  Delay1 : Delay  Commented=on  DelayLength=Delay_step
  Demux5 : Demux  Commented=on  Outputs=6
  Demux6 : Demux  Commented=on  Outputs=6
  Gain1 : Gain  Gain=1e-3
  Goto5 : Goto  Commented=on  GotoTag=beta_y_env_F_L  TagVisibility=global
  Goto6 : Goto  Commented=on  GotoTag=w_env_F_L  TagVisibility=global
  MATLAB Function2 : MATLAB Function  TreatAsAtomicUnit=on
  MATLAB Function3 : MATLAB Function  TreatAsAtomicUnit=on
  MATLAB Function6 : MATLAB Function  TreatAsAtomicUnit=on
  Terminator{1..7,20..22} (10 alike) : Terminator  Commented=on
  To Workspace : ToWorkspace  VariableName=roadprofile_rear_plot  SaveFormat=Timeseries  SampleTime=-1
  X(i)1 : MATLAB Function  TreatAsAtomicUnit=on
  Z_road with noise2 : Lookup_n-D  Commented=on  NumberOfTableDimensions=1  BreakpointsForDimension1=test_distance  Table=road_with_noise  InterpMethod=Flat  InternalRulePriority=Speed  RndMeth=Simplest
  Z_road1 : Lookup_n-D  NumberOfTableDimensions=1  BreakpointsForDimension1=test_distance  Table=road_profile  InterpMethod=Flat  InternalRulePriority=Speed  RndMeth=Simplest
  Z_road2 : Lookup_n-D  NumberOfTableDimensions=1  BreakpointsForDimension1=test_distance  Table=road_profile  InterpMethod=Flat  InternalRulePriority=Speed  RndMeth=Simplest
  w : Outport
  beta_y : Outport  Port=2
  mu_prev : Outport  Port=3
  wires:
  Demux6/1 -> Goto5/1
  Demux6/5 -> Terminator7/1
  Demux6/2 -> Terminator5/1
  Demux6/3 -> Terminator6/1
  Demux6/6 -> Terminator3/1
  Demux6/4 -> Terminator4/1
  Demux5/4 -> Terminator2/1
  Demux5/5 -> Terminator22/1
  Demux5/6 -> Terminator1/1
  Demux5/3 -> Terminator21/1
  Demux5/2 -> Terminator20/1
  Demux5/1 -> Goto6/1
  MATLAB Function3/2(beta_y) -> beta_y/1, Demux6/1
  x_u_dot/1 -> X(i)1/2(x_u_dot_current)
  MATLAB Function6/1(X_road) -> Z_road1/1
  Z_road1/1 -> Gain1/1
  MATLAB Function3/1(w) -> Demux5/1, w/1
  Gain1/1 -> MATLAB Function2/1(z_road)
  X(i)1/1(X_i) -> 1-D Lookup Table/1, MATLAB Function6/1(X_i)  "X(i)"
  MATLAB Function2/2(Z_er) -> MATLAB Function3/2(Z_er)
  MATLAB Function2/1(Z_ef) -> MATLAB Function3/1(Z_ef)
  Z_road2/1 -> To Workspace/1
  x_u/1 -> X(i)1/1(X_u_current), Z_road2/1
  1-D Lookup Table/1 -> mu_prev/1

== system Full_Car_Model/CONTROLLER REAR LEFT/Rule based/Flag ==
  Measurement data : Inport
  mu_prev : Inport  Port=2
  Add : Sum
  Bus Selector : BusSelector  OutputSignals=Accelerations.x_b_ddot
  Constant : Constant  Value=0.5*data.m_total*data.g*data.a/data.L
  Gain : Gain  Gain=0.5*data.m_total*data.hg/data.L
  Gain1 : Gain  Gain=0.6
  GreaterThan : RelationalOperator  Operator=>  OutDataTypeStr=boolean  RndMeth=Simplest  InputSameDT=off
  Memory : Memory
  OR : Logic  Operator=OR  Inputs=1  IconShape=distinctive  AllPortsSameDT=off  OutDataTypeStr=boolean
  Product : Product
  Flag : Outport
  wires:
  Constant/1 -> Add/1
  Bus Selector/1 -> Memory/1  "<x_b_ddot>"
  [Ft_req_R] -> GreaterThan/1
  Gain/1 -> Add/2
  Add/1 -> Product/1
  Measurement data/1 -> Bus Selector/1
  GreaterThan/1 -> OR/1
  Product/1 -> Gain1/1
  Memory/1 -> Gain/1
  mu_prev/1 -> Product/2
  Gain1/1 -> GreaterThan/2
  OR/1 -> Flag/1

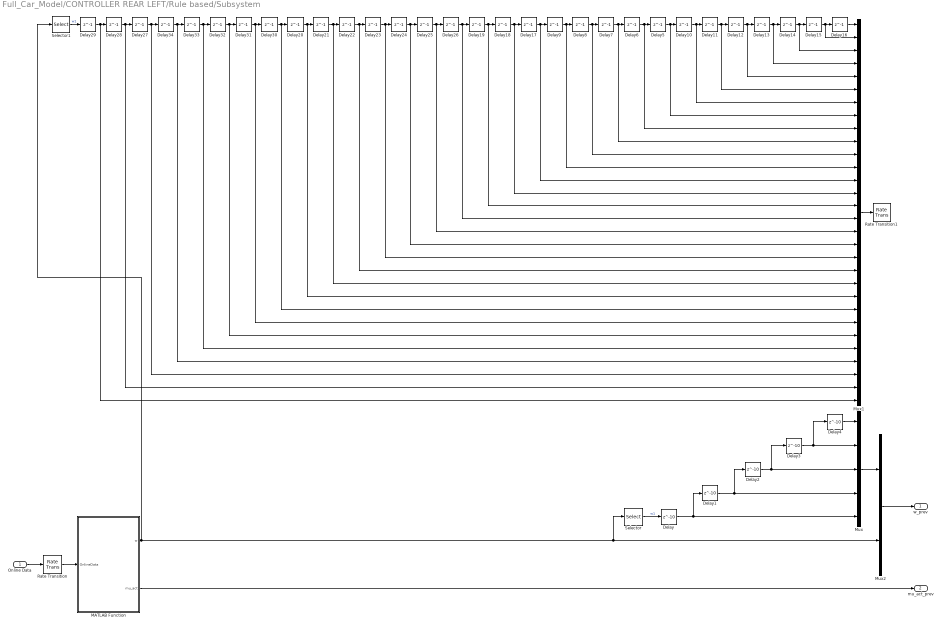
== system Full_Car_Model/CONTROLLER REAR LEFT/Rule based/Subsystem ==
  Online Data : Inport
  Delay{,1..4} (5 alike) : Delay  DelayLength=10
  Delay{5..34} (30 alike) : Delay  DelayLength=1
  MATLAB Function : MATLAB Function  TreatAsAtomicUnit=on
  Mux : Mux  Inputs=5
  Mux1 : Mux  Inputs=30
  Mux2 : Mux  Inputs=2
  Rate Transition : RateTransition  OutPortSampleTime=Ts(2)
  Rate Transition1 : RateTransition  OutPortSampleTime=Ts(2)
  Selector : Selector  NumberOfDimensions=2  InputPortWidth=1  IndexOptions=Index vector (dialog),Select all  Indices=1,1  OutputSizes=1,1
  Selector1 : Selector  NumberOfDimensions=2  InputPortWidth=1  IndexOptions=Index vector (dialog),Select all  Indices=1,1  OutputSizes=1,1
  w_prev : Outport
  mu_act_prev : Outport  Port=2
  wires:
  MATLAB Function/1(w) -> Mux2/2, Selector/1, Selector1/1
  MATLAB Function/2(mu_act) -> mu_act_prev/1
  Mux1/1 -> Rate Transition1/1
  Rate Transition/1 -> MATLAB Function/1(OnlineData)
  Mux2/1 -> w_prev/1
  Delay4/1 -> Mux/1
  Delay3/1 -> Delay4/1, Mux/2
  Delay2/1 -> Delay3/1, Mux/3
  Delay1/1 -> Mux/4, Delay2/1
  Delay/1 -> Mux/5, Delay1/1
  Selector/1 -> Delay/1  "w1"
  Online Data/1 -> Rate Transition/1
  Delay5/1 -> Mux1/8, Delay10/1
  Selector1/1 -> Delay29/1  "w1"
  Delay10/1 -> Mux1/7, Delay11/1
  Delay11/1 -> Mux1/6, Delay12/1
  Delay12/1 -> Mux1/5, Delay13/1
  Delay13/1 -> Mux1/4, Delay14/1
  Delay14/1 -> Mux1/3, Delay15/1
  Delay15/1 -> Mux1/2, Delay16/1
  Delay16/1 -> Mux1/1
  Delay6/1 -> Mux1/9, Delay5/1
  Delay7/1 -> Mux1/10, Delay6/1
  Delay8/1 -> Delay7/1, Mux1/11
  Delay9/1 -> Mux1/12, Delay8/1
  Delay17/1 -> Mux1/13, Delay9/1
  Delay18/1 -> Mux1/14, Delay17/1
  Delay19/1 -> Delay18/1, Mux1/15
  Delay26/1 -> Mux1/16, Delay19/1
  Delay25/1 -> Mux1/17, Delay26/1
  Delay24/1 -> Mux1/18, Delay25/1
  Delay22/1 -> Mux1/20, Delay23/1
  Delay34/1 -> Mux1/27, Delay33/1
  Delay33/1 -> Mux1/26, Delay32/1
  Delay31/1 -> Mux1/24, Delay30/1
  Delay32/1 -> Mux1/25, Delay31/1
  Delay30/1 -> Mux1/23, Delay20/1
  Delay28/1 -> Mux1/29, Delay27/1
  Delay27/1 -> Mux1/28, Delay34/1
  Delay23/1 -> Mux1/19, Delay24/1
  Delay21/1 -> Mux1/21, Delay22/1
  Delay29/1 -> Mux1/30, Delay28/1
  Delay20/1 -> Mux1/22, Delay21/1
  Mux/1 -> Mux2/1

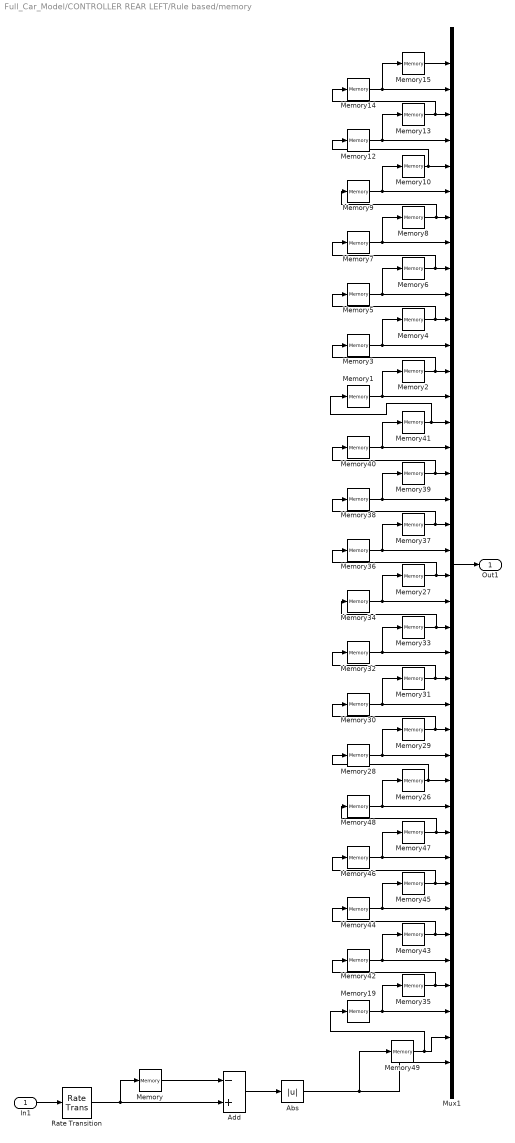
== system Full_Car_Model/CONTROLLER REAR LEFT/Rule based/memory ==
  In1 : Inport
  Abs : Abs  SaturateOnIntegerOverflow=off
  Add : Sum  Inputs=-+
  Memory{,1..10,12..15,19,26..49} (40 alike) : Memory  InheritSampleTime=on
  Mux1 : Mux  Inputs=40
  Rate Transition : RateTransition  OutPortSampleTime=Ts(2)
  Out1 : Outport
  wires:
  Abs/1 -> Mux1/40, Memory49/1
  Memory49/1 -> Mux1/39, Memory19/1
  Memory19/1 -> Memory35/1, Mux1/38
  Memory47/1 -> Memory48/1, Mux1/31
  Memory42/1 -> Memory43/1, Mux1/36
  Memory44/1 -> Memory45/1, Mux1/34
  Memory43/1 -> Memory44/1, Mux1/35
  Memory33/1 -> Memory34/1, Mux1/23
  Memory46/1 -> Memory47/1, Mux1/32
  Memory32/1 -> Memory33/1, Mux1/24
  Memory38/1 -> Memory39/1, Mux1/18
  Memory48/1 -> Memory26/1, Mux1/30
  Memory45/1 -> Memory46/1, Mux1/33
  Memory30/1 -> Memory31/1, Mux1/26
  Memory26/1 -> Memory28/1, Mux1/29
  Memory37/1 -> Memory38/1, Mux1/19
  Memory29/1 -> Memory30/1, Mux1/27
  Memory31/1 -> Memory32/1, Mux1/25
  Memory27/1 -> Memory36/1, Mux1/21
  Memory28/1 -> Memory29/1, Mux1/28
  Memory34/1 -> Memory27/1, Mux1/22
  Memory40/1 -> Memory41/1, Mux1/16
  Memory41/1 -> Mux1/15, Memory1/1
  Memory39/1 -> Memory40/1, Mux1/17
  Memory35/1 -> Memory42/1, Mux1/37
  Memory36/1 -> Memory37/1, Mux1/20
  Add/1 -> Abs/1
  In1/1 -> Rate Transition/1
  Memory/1 -> Add/1
  Rate Transition/1 -> Add/2, Memory/1
  Memory14/1 -> Memory15/1, Mux1/2
  Memory12/1 -> Memory13/1, Mux1/4
  Memory15/1 -> Mux1/1
  Memory13/1 -> Memory14/1, Mux1/3
  Memory10/1 -> Mux1/5, Memory12/1
  Memory9/1 -> Memory10/1, Mux1/6
  Memory8/1 -> Memory9/1, Mux1/7
  Memory7/1 -> Memory8/1, Mux1/8
  Memory6/1 -> Memory7/1, Mux1/9
  Memory5/1 -> Memory6/1, Mux1/10
  Memory4/1 -> Mux1/11, Memory5/1
  Memory3/1 -> Memory4/1, Mux1/12
  Memory2/1 -> Mux1/13, Memory3/1
  Memory1/1 -> Memory2/1, Mux1/14
  Mux1/1 -> Out1/1

== system Full_Car_Model/CONTROLLER REAR RIGHT/RL_weights/Subsystem2 ==
  Online Data : Inport
  Delay : Delay  Commented=on  DelayLength=1  SampleTime=Ts(2)
  MATLAB Function : MATLAB Function  TreatAsAtomicUnit=on
  Memory{,1..4} (5 alike) : Memory  InheritSampleTime=on
  Mux : Mux  Inputs=5
  Mux2 : Mux  Inputs=2
  Selector : Selector  NumberOfDimensions=2  InputPortWidth=1  IndexOptions=Index vector (dialog),Select all  Indices=1,1  OutputSizes=1,1
  Selector1 : Selector  NumberOfDimensions=2  InputPortWidth=1  IndexOptions=Index vector (dialog),Select all  Indices=1,1  OutputSizes=1,1
  w_prev : Outport
  mu_act_prev : Outport  Port=2
  sigma_ref_act : Outport  Port=3
  wires:
  Online Data/1 -> MATLAB Function/1(OnlineData)
  MATLAB Function/1(w) -> Mux2/2, Selector/1
  Selector/1 -> Memory/1  "w1"
  Memory/1 -> Memory1/1, Mux/5
  Memory1/1 -> Memory2/1, Mux/4
  Memory2/1 -> Memory3/1, Mux/3
  Memory3/1 -> Memory4/1, Mux/2
  Memory4/1 -> Mux/1
  Mux/1 -> Mux2/1
  Mux2/1 -> w_prev/1
  MATLAB Function/2(mu_act) -> mu_act_prev/1
  MATLAB Function/3(sigma_ref) -> Selector1/1
  Selector1/1 -> sigma_ref_act/1

== system Full_Car_Model/CONTROLLER REAR RIGHT/ROAD PREVIEW/Time-based Road Preview ==
  note: Absolute longitudinal wheel position along t_h
      | (assuming contant speed along t_h)
  x_u : Inport
  x_u_dot : Inport  Port=2
  1-D Lookup Table : Lookup_n-D  NumberOfTableDimensions=1  BreakpointsForDimension1=mu_distance  Table=mu_road  InternalRulePriority=Speed  RndMeth=Simplest
  Delay1 : Delay  Commented=on  DelayLength=Delay_step
  Demux5 : Demux  Commented=on  Outputs=6
  Demux6 : Demux  Commented=on  Outputs=6
  Gain1 : Gain  Gain=1e-3
  Goto5 : Goto  Commented=on  GotoTag=beta_y_env_F_L  TagVisibility=global
  Goto6 : Goto  Commented=on  GotoTag=w_env_F_L  TagVisibility=global
  MATLAB Function2 : MATLAB Function  TreatAsAtomicUnit=on
  MATLAB Function3 : MATLAB Function  TreatAsAtomicUnit=on
  MATLAB Function6 : MATLAB Function  TreatAsAtomicUnit=on
  Terminator{1..7,20..22} (10 alike) : Terminator  Commented=on
  X(i)1 : MATLAB Function  TreatAsAtomicUnit=on
  Z_road with noise2 : Lookup_n-D  Commented=on  NumberOfTableDimensions=1  BreakpointsForDimension1=test_distance  Table=road_with_noise  InterpMethod=Flat  InternalRulePriority=Speed  RndMeth=Simplest
  Z_road1 : Lookup_n-D  NumberOfTableDimensions=1  BreakpointsForDimension1=test_distance  Table=road_profile  InterpMethod=Flat  InternalRulePriority=Speed  RndMeth=Simplest
  w : Outport
  beta_y : Outport  Port=2
  mu_prev : Outport  Port=3
  wires:
  Demux6/1 -> Goto5/1
  Demux6/5 -> Terminator7/1
  Demux6/2 -> Terminator5/1
  Demux6/3 -> Terminator6/1
  Demux6/6 -> Terminator3/1
  Demux6/4 -> Terminator4/1
  Demux5/4 -> Terminator2/1
  Demux5/5 -> Terminator22/1
  Demux5/6 -> Terminator1/1
  Demux5/3 -> Terminator21/1
  Demux5/2 -> Terminator20/1
  Demux5/1 -> Goto6/1
  MATLAB Function3/2(beta_y) -> beta_y/1, Demux6/1
  x_u_dot/1 -> X(i)1/2(x_u_dot_current)
  x_u/1 -> X(i)1/1(X_u_current)
  MATLAB Function6/1(X_road) -> Z_road1/1
  Z_road1/1 -> Gain1/1
  MATLAB Function3/1(w) -> Demux5/1, w/1
  Gain1/1 -> MATLAB Function2/1(z_road)
  X(i)1/1(X_i) -> 1-D Lookup Table/1, MATLAB Function6/1(X_i)  "X(i)"
  1-D Lookup Table/1 -> mu_prev/1
  MATLAB Function2/2(Z_er) -> MATLAB Function3/2(Z_er)
  MATLAB Function2/1(Z_ef) -> MATLAB Function3/1(Z_ef)

== system Full_Car_Model/CONTROLLER REAR RIGHT/Rule based/Flag ==
  Measurement data : Inport
  mu_prev : Inport  Port=2
  Add : Sum
  Bus Selector : BusSelector  OutputSignals=Accelerations.x_b_ddot
  Constant : Constant  Value=0.5*data.m_total*data.g*data.a/data.L
  Gain : Gain  Gain=0.5*data.m_total*data.hg/data.L
  Gain1 : Gain  Gain=0.6
  GreaterThan : RelationalOperator  Operator=>  OutDataTypeStr=boolean  RndMeth=Simplest  InputSameDT=off
  Memory : Memory
  OR : Logic  Operator=OR  Inputs=1  IconShape=distinctive  AllPortsSameDT=off  OutDataTypeStr=boolean
  Product : Product
  Scope : Scope  NumInputPorts=3
  Flag : Outport
  wires:
  Constant/1 -> Add/1
  Bus Selector/1 -> Memory/1  "<x_b_ddot>"
  [Ft_req_R] -> Scope/1, GreaterThan/1
  Gain/1 -> Add/2
  Add/1 -> Product/1
  Measurement data/1 -> Bus Selector/1
  GreaterThan/1 -> Scope/3, OR/1
  Product/1 -> Gain1/1
  Memory/1 -> Gain/1
  mu_prev/1 -> Product/2
  Gain1/1 -> Scope/2, GreaterThan/2
  OR/1 -> Flag/1
